simulink model "electric_tractor"  (R2024b)
settings: Solver=ode4  StartTime=0.0  StopTime=60  FixedStep=0.001  RelTol=1e-3
values from neighbouring files (symbols this model uses):
  A = 2.5    [init.m]
  C_d = 0.80    (= 0.8)    [init.m]
  eta_drive = 0.95    [init.m]
  eta_motor = 0.90    (= 0.9)    [init.m]
  F_grade = P.m * P.g * sin(theta_rad)    [genetic_fuzzy_optimizer.m]    (also in init.m = m * g * sin(theta_rad))
  F_implement = sigma * d_impl * w_impl    (= 0)    [init.m]
  F_roll = mu_rr * P.m * P.g * cos(theta_rad)    [genetic_fuzzy_optimizer.m]    (also in init.m = mu_rr * m * g * cos(theta_rad))
  G_r = 30    [init.m]
  lambda_f = 0.15    [init.m]
  m = 2470    [init.m]
  P_poles = 6    [init.m]
  r_wheel = 0.72    [init.m]
  rho_air = 1.225    [init.m]
  SoC_0 = 1.0    (= 1)    [init.m]
  SoC_min = 0.20    (= 0.2)    [init.m]
  T_rated = 200    [init.m]
  tau_m = 0.05    [init.m]
  v_ref = v_ss    [compare_original_vs_ga.m]    (also in genetic_fuzzy_optimizer.m = P.modes(mode_idx, 1); init.m = 3.33333333333)
libraries: fuzblock x1, slpidlib x1
settings Model: Creator=USER  LastModifiedBy=USER

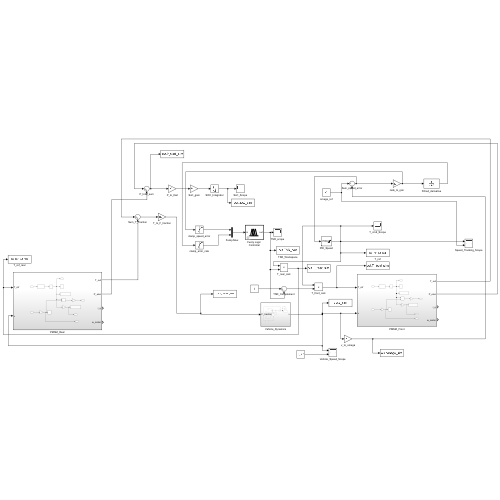
[thumbnail: Simulink's stored preview of the top-level diagram]
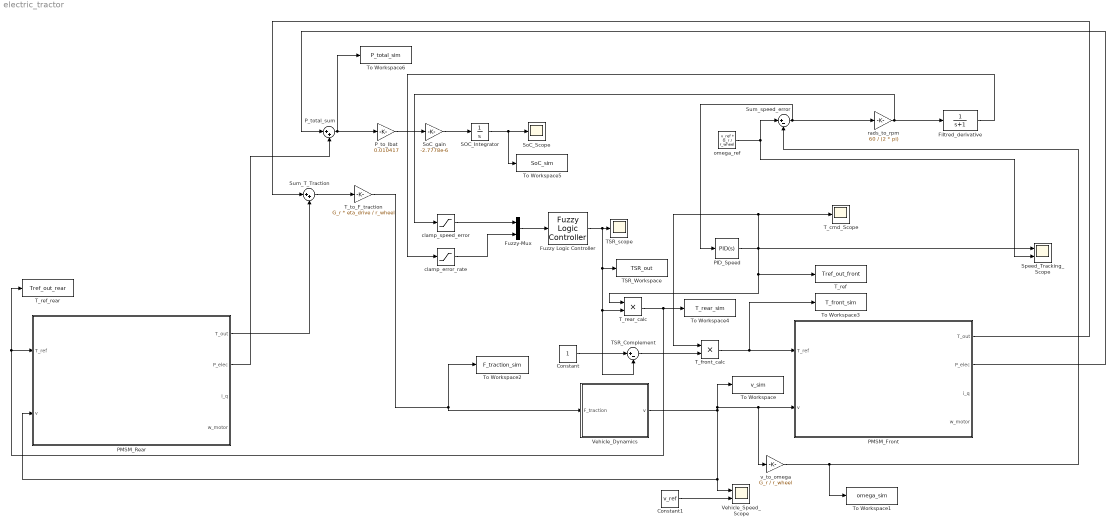
== system electric_tractor ==
  Constant : Constant
  Constant1 : Constant  Value=v_ref
  Filtred_derivative : TransferFcn  Denominator=[1 1]
  Fuzzy Logic Controller : fuzblock/Fuzzy Logic  Controller  FIS='tractor_torque_controller.fis'  OutputSampleNumber=101  DataType=double  FuzzifiedInputs=off  RuleFiringStrengths=off  RuleOutputs=off  AggregatedOutputs=off  SimulateUsing=Interpreted execution  OutOfRangeInputValueMessage=warning  NoRuleFiredMessage=warning  EmptyOutputFuzzySetMessage=warning
  Fuzzy-Mux : Mux  Inputs=2
  PID_Speed : slpidlib/PID Controller  Controller=PID  Form=Parallel  TimeDomain=Continuous-time  UseExternalTs=off  SampleTime=-1  IntegratorMethod=Forward Euler  FilterMethod=Forward Euler  ControllerParametersSource=internal  P=3.90  I=10.83  UseKiTs=off  D=0.35  UseExternalDerivativeSource=off  N=100  UseFilter=on  TunerSelectOption=Transfer Function Based (PID Tuner App)  InitialConditionSource=internal  InitialConditionForIntegrator=0  InitialConditionForFilter=0  DifferentiatorICPrevScaledInput=0  ExternalReset=none  TrackingMode=off  Kt=1  LimitOutput=on  SatLimitsSource=internal  UpperSaturationLimit=400  LowerSaturationLimit=0  LinearizeAsGain=on  AntiWindupMode=clamping  Kb=1  LimitIntegrator=off  UpperIntegratorSaturationLimit=inf  LowerIntegratorSaturationLimit=-inf  POutMin=[]  POutMax=[]  IOutMin=[]  IOutMax=[]  DOutMin=[]  DOutMax=[]  NOutMin=[]  NOutMax=[]  SumOutMin=[]  SumOutMax=[]  SaturationOutMin=[]  SaturationOutMax=[]  PParamMin=[]  PParamMax=[]  IParamMin=[]  IParamMax=[]  DParamMin=[]  DParamMax=[]  NParamMin=[]  NParamMax=[]  KbParamMin=[]  KbParamMax=[]  KtParamMin=[]  KtParamMax=[]  KbOutMin=[]  KbOutMax=[]  KtOutMin=[]  KtOutMax=[]  IntegratorOutMin=[]  IntegratorOutMax=[]  FilterOutMin=[]  FilterOutMax=[]  SumI1OutMin=[]  SumI1OutMax=[]  SumI2OutMin=[]  SumI2OutMax=[]  SumI3OutMin=[]  SumI3OutMax=[]  SumI4OutMin=[]  SumI4OutMax=[]  SumDOutMin=[]  SumDOutMax=[]  DifferentiatorOutMin=[]  DifferentiatorOutMax=[]  FilterDiffOutCoefMin=[]  FilterDiffOutCoefMax=[]  ReciprocalOutMin=[]  ReciprocalOutMax=[]  SumDenOutMin=[]  SumDenOutMax=[]  SumNumOutMin=[]  SumNumOutMax=[]  DivideOutMin=[]  DivideOutMax=[]  UdiffTsProdOutMin=[]  UdiffTsProdOutMax=[]  NTsProdOutMin=[]  NTsProdOutMax=[]  UintegralTsProdOutMin=[]  UintegralTsProdOutMax=[]  UngainTsProdOutMin=[]  UngainTsProdOutMax=[]  ClampingZeroOutDataTypeStr=Inherit: Inherit via back propagation  ClampingZeroOutMin=[]  ClampingZeroOutMax=[]  FilterDenConstantOutDataTypeStr=Inherit: Inherit via back propagation  FilterDenConstantOutMin=[]  FilterDenConstantOutMax=[]  PCopyOutDataTypeStr=Inherit: Inherit via back propagation  PCopyOutMin=[]  PCopyOutMax=[]  NCopyOutDataTypeStr=Inherit: Inherit via back propagation  NCopyOutMin=[]  NCopyOutMax=[]  IntegratorContinuousStateAttributes=''  IntegratorStateMustResolveToSignalObject=off  IntegratorRTWStateStorageClass=Auto  FilterContinuousStateAttributes=''  FilterStateMustResolveToSignalObject=off  FilterRTWStateStorageClass=Auto  ParallelPVariant=InternalParameters  IdealPVariant=Disabled  IVariant=InternalParameters  DVariant=InternalParameters  IntegratorVariant=Continuous  SatVariant=Enabled  AWVariant=ContClampingParallel  PCopyVariant=Disabled  TRVariant=Disabled  FdbkBlocksVariant=Forward  IdealPFdbkVariant=Disabled  SatFdbkVariant=Disabled  DerivativeFilterVariant=ContFilter  NVariant=InternalParameters  NCopyVariant=Disabled  FilterICVariant=InternalICsFilter  IntegratorICVariant=InternalICs  ExternalResetVariant=Disabled  TRSumVariant=Passthrough  SumFdbkVariant=Disabled  SumVariant=Sum_PID  TsampFilterVariant=InternalTs  TsampNgainVariant=Passthrough  TsampIntegralVariant=Disabled_SignalSpec  ExternalSaturationOutDataTypeStr=Inherit: Same as second input  DerivativeSourceVariant=ErrorSignal  PreIntVariant=InternalPreInt
  PMSM_Front : Subsystem
  PMSM_Rear : Subsystem
  P_to_Ibat : Gain  Gain=0.010417
  P_total_sum : Sum  Inputs=|++
  SOC_Integrator : Integrator  InitialCondition=SoC_0  LimitOutput=on  UpperSaturationLimit=1  LowerSaturationLimit=SoC_min
  SoC_Scope : Scope
  SoC_gain : Gain  Gain=-2.7778e-6
  Speed_Tracking_Scope : Scope  NumInputPorts=2
  Sum_T_Traction : Sum  Inputs=|++
  Sum_speed_error : Sum  Inputs=|+-
  TSR_Complement : Sum  Inputs=|+-
  TSR_Workspace : ToWorkspace  VariableName=TSR_out  SampleTime=-1
  TSR_scope : Scope
  T_cmd_Scope : Scope
  T_front_calc : Product
  T_rear_calc : Product
  T_ref : ToWorkspace  VariableName=Tref_out_front  SampleTime=-1
  T_ref_rear : ToWorkspace  VariableName=Tref_out_rear  SampleTime=-1
  T_to_F_traction : Gain  Gain=G_r * eta_drive / r_wheel
  To Workspace : ToWorkspace  VariableName=v_sim  SampleTime=-1
  To Workspace1 : ToWorkspace  VariableName=omega_sim  SampleTime=-1
  To Workspace2 : ToWorkspace  VariableName=F_traction_sim  SampleTime=-1
  To Workspace3 : ToWorkspace  VariableName=T_front_sim  SampleTime=-1
  To Workspace4 : ToWorkspace  VariableName=T_rear_sim  SampleTime=-1
  To Workspace5 : ToWorkspace  VariableName=SoC_sim  SampleTime=-1
  To Workspace6 : ToWorkspace  VariableName=P_total_sim  SampleTime=-1
  Vehicle_Dynamics : Subsystem
  Vehicle_Speed_Scope : Scope  NumInputPorts=2
  clamp_error_rate : Saturate  UpperLimit=5  LowerLimit=-5
  clamp_speed_error : Saturate  UpperLimit=10  LowerLimit=-10
  omega_ref : Constant  Value=v_ref * G_r / r_wheel
  rads_to_rpm : Gain  Gain=60 / (2 * pi)
  v_to_omega : Gain  Gain=G_r / r_wheel
  wires:
  omega_ref/1 -> Speed_Tracking_Scope/2, Sum_speed_error/1
  PID_Speed/1 -> T_front_calc/1, T_cmd_Scope/1, T_rear_calc/1, T_ref/1, Speed_Tracking_Scope/1
  Fuzzy Logic Controller/1 -> TSR_Workspace/1, T_rear_calc/2, TSR_Complement/2, TSR_scope/1
  T_front_calc/1 -> To Workspace3/1, PMSM_Front/1(T_ref)
  T_rear_calc/1 -> To Workspace4/1, T_ref_rear/1, PMSM_Rear/1(T_ref)
  Constant/1 -> TSR_Complement/1
  rads_to_rpm/1 -> clamp_speed_error/1, Filtred_derivative/1
  Fuzzy-Mux/1 -> Fuzzy Logic Controller/1
  clamp_speed_error/1 -> Fuzzy-Mux/1
  clamp_error_rate/1 -> Fuzzy-Mux/2
  Filtred_derivative/1 -> clamp_error_rate/1
  PMSM_Front/1(T_out) -> Sum_T_Traction/1
  PMSM_Rear/1(T_out) -> Sum_T_Traction/2
  SoC_gain/1 -> SOC_Integrator/1
  Vehicle_Dynamics/1(v) -> To Workspace/1, v_to_omega/1, PMSM_Front/2(v), Vehicle_Speed_Scope/1, PMSM_Rear/2(v)
  Sum_T_Traction/1 -> T_to_F_traction/1
  T_to_F_traction/1 -> To Workspace2/1, Vehicle_Dynamics/1(F_traction)
  PMSM_Front/2(P_elec) -> P_total_sum/1
  PMSM_Rear/2(P_elec) -> P_total_sum/2
  P_total_sum/1 -> P_to_Ibat/1, To Workspace6/1
  P_to_Ibat/1 -> SoC_gain/1
  SOC_Integrator/1 -> To Workspace5/1, SoC_Scope/1
  v_to_omega/1 -> To Workspace1/1, Sum_speed_error/2
  TSR_Complement/1 -> T_front_calc/2
  Constant1/1 -> Vehicle_Speed_Scope/2
  Sum_speed_error/1 -> PID_Speed/1, rads_to_rpm/1

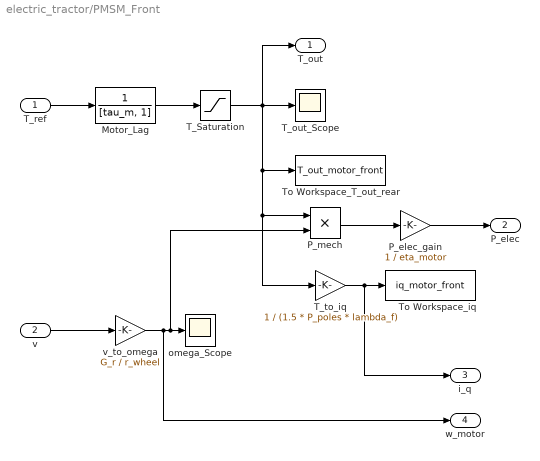
== system electric_tractor/PMSM_Front ==
  T_ref : Inport
  v : Inport  Port=2
  Motor_Lag : TransferFcn  Denominator=[tau_m, 1]
  P_elec_gain : Gain  Gain=1 / eta_motor
  P_mech : Product
  T_Saturation : Saturate  UpperLimit=T_rated  LowerLimit=0
  T_out_Scope : Scope
  T_to_iq : Gain  Gain=1 / (1.5 * P_poles * lambda_f)
  To Workspace_T_out_rear : ToWorkspace  VariableName=T_out_motor_front  SampleTime=-1
  To Workspace_iq : ToWorkspace  VariableName=iq_motor_front  SampleTime=-1
  omega_Scope : Scope
  v_to_omega : Gain  Gain=G_r / r_wheel
  T_out : Outport
  P_elec : Outport  Port=2
  i_q : Outport  Port=3
  w_motor : Outport  Port=4
  wires:
  P_mech/1 -> P_elec_gain/1
  T_to_iq/1 -> To Workspace_iq/1, i_q/1
  v_to_omega/1 -> P_mech/2, omega_Scope/1, w_motor/1
  Motor_Lag/1 -> T_Saturation/1
  T_Saturation/1 -> T_out_Scope/1, To Workspace_T_out_rear/1, P_mech/1, T_to_iq/1, T_out/1
  v/1 -> v_to_omega/1
  T_ref/1 -> Motor_Lag/1
  P_elec_gain/1 -> P_elec/1

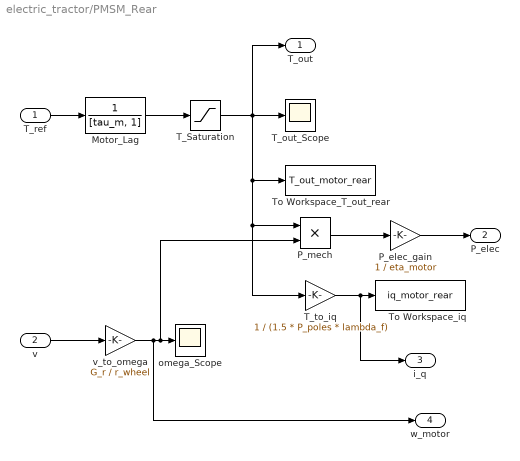
== system electric_tractor/PMSM_Rear ==
  T_ref : Inport
  v : Inport  Port=2
  Motor_Lag : TransferFcn  Denominator=[tau_m, 1]
  P_elec_gain : Gain  Gain=1 / eta_motor
  P_mech : Product
  T_Saturation : Saturate  UpperLimit=T_rated  LowerLimit=0
  T_out_Scope : Scope
  T_to_iq : Gain  Gain=1 / (1.5 * P_poles * lambda_f)
  To Workspace_T_out_rear : ToWorkspace  VariableName=T_out_motor_rear  SampleTime=-1
  To Workspace_iq : ToWorkspace  VariableName=iq_motor_rear  SampleTime=-1
  omega_Scope : Scope
  v_to_omega : Gain  Gain=G_r / r_wheel
  T_out : Outport
  P_elec : Outport  Port=2
  i_q : Outport  Port=3
  w_motor : Outport  Port=4
  wires:
  P_mech/1 -> P_elec_gain/1
  T_to_iq/1 -> i_q/1, To Workspace_iq/1
  v_to_omega/1 -> P_mech/2, omega_Scope/1, w_motor/1
  Motor_Lag/1 -> T_Saturation/1
  T_Saturation/1 -> T_out_Scope/1, To Workspace_T_out_rear/1, P_mech/1, T_to_iq/1, T_out/1
  P_elec_gain/1 -> P_elec/1
  T_ref/1 -> Motor_Lag/1
  v/1 -> v_to_omega/1

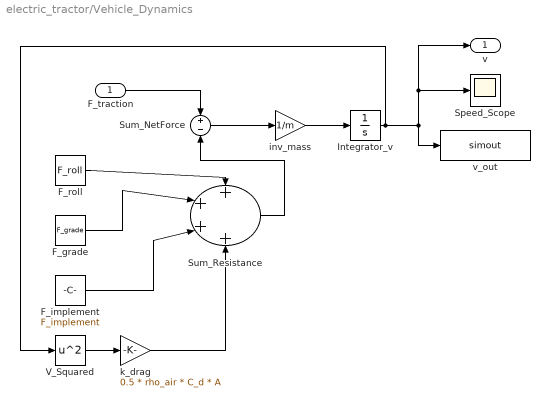
== system electric_tractor/Vehicle_Dynamics ==
  F_traction : Inport
  F_grade : Constant  Value=F_grade
  F_implement : Constant  Value=F_implement
  F_roll : Constant  Value=F_roll
  Integrator_v : Integrator  LimitOutput=on  LowerSaturationLimit=0
  Speed_Scope : Scope
  Sum_NetForce : Sum  Inputs=+-
  Sum_Resistance : Sum  Inputs=++++
  V_Squared : Math  Operator=square
  inv_mass : Gain  Gain=1/m
  k_drag : Gain  Gain=0.5 * rho_air * C_d * A
  v_out : ToWorkspace  VariableName=simout  SaveFormat=Timeseries  SampleTime=-1
  v : Outport
  wires:
  Sum_NetForce/1 -> inv_mass/1
  V_Squared/1 -> k_drag/1
  Integrator_v/1 -> V_Squared/1, Speed_Scope/1, v/1, v_out/1
  Sum_Resistance/1 -> Sum_NetForce/2
  inv_mass/1 -> Integrator_v/1
  F_implement/1 -> Sum_Resistance/3
  k_drag/1 -> Sum_Resistance/4
  F_roll/1 -> Sum_Resistance/1
  F_grade/1 -> Sum_Resistance/2
  F_traction/1 -> Sum_NetForce/1
